simulink model "QD2_DroneStack_MPC"  (R2023a)
settings: Solver=ode1  StartTime=0.0  StopTime=inf  FixedStep=1/1000  RelTol=1e-3  EnableMultiTasking=on
InitFcn:
  | % QD2_DroneStack_MPC: rutas de la librería qd2_* y del mapeo de motores
  | qd2_d = fileparts(get_param(bdroot, 'FileName'));
  | for qd2_k = 1:4
  |     if exist(fullfile(qd2_d, 'lib', 'qd2_params.m'), 'file'), break; end
  |     qd2_d = fileparts(qd2_d);
  | end
  | addpath(fullfile(qd2_d, 'lib'));
  | addpath(fullfile(qd2_d, 'equipo2_original'));
  | clear qd2_d qd2_k
  | Motor_Mapping_7_Inch
model workspace (MAT data in the model file):
  target_system = 1
undefined symbols (not defined in the file): _Commander, _QDrone2, _Stabilizer, datetime, HIL, KT, lf, log_, m, Motor_Matrix, n, qc_get_step_size, s, saved_data
libraries: quarc_library x94, simulink x27, simulink_extras x9
(part 3 of 5)

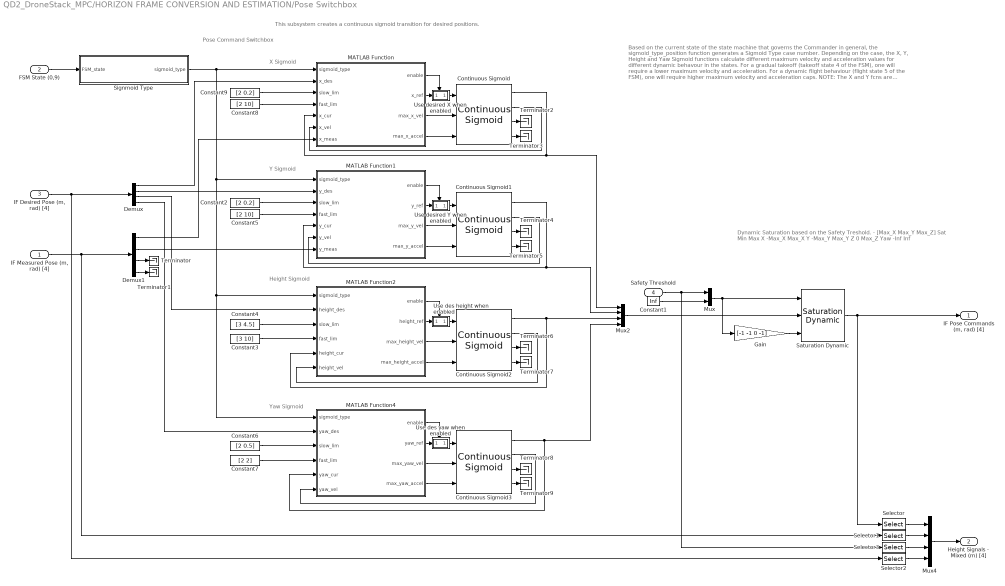
== system QD2_DroneStack_MPC/HORIZON FRAME CONVERSION AND ESTIMATION/Pose Switchbox ==
  note: Dynamic Saturation based on the Safety Treshold. - [Max_X Max_Y Max_Z]
      |
      | Sat Min Max
      | X -Max_X Max_X
      | Y -Max_Y Max_Y
      | Z 0 Max_Z
      | Yaw -Inf Inf
  note: Based on the current state of the state machine that governs the Commander in general,
      | the sigmoid_type_position function generates a Sigmoid Type case number. Depending on
      | the case, the X, Y, Height and Yaw Sigmoid functions calculate different maximum velocity
      | and acceleration values for different dynamic behavour in the states.
      |
      | For a gradual takeoff (takeoff state 4 of the FSM), one will require a lower maximum velocity
      | and acceleration. For a dynamic flight behaviour (flight state 5 of the FSM), one will require
      | higher maximum velocity and acceleration caps.
      |
      | NOTE: The X and Y fcns are logically identical due to the generally symmetric X and Y behaviour.
      | The Z and Yaw fcns are different.
  note: This subsystem creates a continuous sigmoid transition for desired positions.
  note: Height Sigmoid
  note: Pose Command Switchbox
  note: X Sigmoid
  note: Yaw Sigmoid
  note: Y Sigmoid
  "IF Measured Pose (m, rad) [4]" : Inport
  FSM State (0,9) : Inport  Port=2
  "IF Desired Pose (m, rad) [4]" : Inport  Port=3
  Safety Threshold : Inport  Port=4
  Constant1 : Constant  Value=Inf
  Constant2 : Constant  Value=[2 0.2]
  Constant3 : Constant  Value=[3 10]
  Constant4 : Constant  Value=[3 4.5]
  Constant5 : Constant  Value=[2 10]
  Constant6 : Constant  Value=[2 0.5]
  Constant7 : Constant  Value=[2 2]
  Constant8 : Constant  Value=[2 10]
  Constant9 : Constant  Value=[2 0.2]
  Continuous Sigmoid{,1..3} (4 alike) : quarc_library/Sources/Sigmoids/Continuous Sigmoid  params_source=External (input ports)  max_velocity=2  max_acceleration=10  initial_position=0  initial_velocity=0  hold_off=0.5  input_sample_time=-1  output_sample_time=qc_get_step_size
      settings: SourceProductName=QUARC Targets
  Demux : Demux
  Demux1 : Demux
  Gain : Gain  Gain=[-1 -1 0 -1]
  MATLAB Function : MATLAB Function  TreatAsAtomicUnit=on
  MATLAB Function1 : MATLAB Function  TreatAsAtomicUnit=on
  MATLAB Function2 : MATLAB Function  TreatAsAtomicUnit=on
  MATLAB Function4 : MATLAB Function  TreatAsAtomicUnit=on
  Mux : Mux  Inputs=2
  Mux2 : Mux
  Mux4 : Mux
  Saturation Dynamic : simulink/Discontinuities/Saturation Dynamic  OutMin=[]  OutMax=[]  OutDataTypeStr=Inherit: Same as second input  OutDataType=fixdt(1, 16)  OutScaling=2^-10  DoSatur=off
  Selector : Selector  InputPortWidth=4  IndexOptions=Index vector (dialog)  Indices=[3]  OutputSizes=1
  Selector1 : Selector  InputPortWidth=4  IndexOptions=Index vector (dialog)  Indices=[3]  OutputSizes=1
  Selector2 : Selector  InputPortWidth=4  IndexOptions=Index vector (dialog)  Indices=[3]  OutputSizes=1
  Selector3 : Selector  InputPortWidth=3  IndexOptions=Index vector (dialog)  Indices=[3]  OutputSizes=1
  Signmoid Type : MATLAB Function  TreatAsAtomicUnit=on
  Terminator{,1..9} (10 alike) : Terminator
  Use des height when enabled : Subsystem  TreatAsAtomicUnit=on
  Use des yaw when enabled : Subsystem  TreatAsAtomicUnit=on
  Use desired X when enabled : Subsystem  TreatAsAtomicUnit=on
  Use desired Y when enabled : Subsystem  TreatAsAtomicUnit=on
  "IF Pose Commands (m, rad) [4]" : Outport  VectorParamsAs1DForOutWhenUnconnected=off
  Height Signals - Mixed (m) [4] : Outport  Port=2  VectorParamsAs1DForOutWhenUnconnected=off
  wires:
  Constant4/1 -> MATLAB Function2/3(slow_lim)
  Constant3/1 -> MATLAB Function2/4(fast_lim)
  Selector/1 -> Mux4/1
  Selector1/1 -> Mux4/2
  Selector2/1 -> Mux4/4
  Selector3/1 -> Mux4/3
  Safety Threshold/1 -> Mux/1, Selector3/1
  Mux/1 -> Saturation Dynamic/1, Gain/1
  Constant1/1 -> Mux/2
  Saturation Dynamic/1 -> "IF Pose Commands (m, rad) [4]"/1, Selector/1
  Mux2/1 -> Saturation Dynamic/2
  Mux4/1 -> Height Signals - Mixed (m) [4]/1
  Gain/1 -> Saturation Dynamic/3
  Demux/2 -> MATLAB Function1/2(y_des)
  Use desired Y when enabled/1(Out1) -> Continuous Sigmoid1/1
  Use desired X when enabled/1(Out1) -> Continuous Sigmoid/1
  MATLAB Function2/3(max_height_vel) -> Continuous Sigmoid2/2
  Continuous Sigmoid3/3 -> Terminator8/1
  Demux1/4 -> Terminator1/1
  MATLAB Function4/1(enable) -> Use des yaw when enabled/Enable
  Use des yaw when enabled/1(Out1) -> Continuous Sigmoid3/1
  Continuous Sigmoid1/2 -> MATLAB Function1/6(y_vel)
  Constant2/1 -> MATLAB Function1/3(slow_lim)
  Constant6/1 -> MATLAB Function4/3(slow_lim)
  Demux1/1 -> MATLAB Function/7(x_meas)
  MATLAB Function1/2(y_ref) -> Use desired Y when enabled/1(h_d (m) [1])
  Demux/3 -> MATLAB Function2/2(height_des)
  Constant7/1 -> MATLAB Function4/4(fast_lim)
  Continuous Sigmoid1/4 -> Terminator5/1
  MATLAB Function1/1(enable) -> Use desired Y when enabled/Enable
  Continuous Sigmoid2/4 -> Terminator7/1
  Demux1/3 -> Terminator/1
  Signmoid Type/1(sigmoid_type) -> MATLAB Function/1(sigmoid_type), MATLAB Function1/1(sigmoid_type), MATLAB Function2/1(sigmoid_type), MATLAB Function4/1(sigmoid_type)
  MATLAB Function/3(max_x_vel) -> Continuous Sigmoid/2
  MATLAB Function2/1(enable) -> Use des height when enabled/Enable
  Constant9/1 -> MATLAB Function/3(slow_lim)
  Continuous Sigmoid2/2 -> MATLAB Function2/6(height_vel)
  Continuous Sigmoid1/1 -> MATLAB Function1/5(y_cur), Mux2/2
  MATLAB Function4/4(max_yaw_accel) -> Continuous Sigmoid3/3
  Demux/1 -> MATLAB Function/2(x_des)
  MATLAB Function1/3(max_y_vel) -> Continuous Sigmoid1/2
  Continuous Sigmoid3/2 -> MATLAB Function4/6(yaw_vel)
  MATLAB Function2/2(height_ref) -> Use des height when enabled/1(h_d (m) [1])
  MATLAB Function/4(max_x_accel) -> Continuous Sigmoid/3
  Use des height when enabled/1(Out1) -> Continuous Sigmoid2/1
  Continuous Sigmoid2/3 -> Terminator6/1
  Demux/4 -> MATLAB Function4/2(yaw_des)
  MATLAB Function1/4(max_y_accel) -> Continuous Sigmoid1/3
  MATLAB Function/1(enable) -> Use desired X when enabled/Enable
  Continuous Sigmoid3/4 -> Terminator9/1
  MATLAB Function4/2(yaw_ref) -> Use des yaw when enabled/1(h_d (m) [1])
  FSM State (0,9)/1 -> Signmoid Type/1(FSM_state)
  MATLAB Function2/4(max_height_accel) -> Continuous Sigmoid2/3
  Continuous Sigmoid/4 -> Terminator3/1
  Continuous Sigmoid/3 -> Terminator2/1
  Continuous Sigmoid/1 -> MATLAB Function/5(x_cur), Mux2/1
  Continuous Sigmoid/2 -> MATLAB Function/6(x_vel)
  MATLAB Function/2(x_ref) -> Use desired X when enabled/1(h_d (m) [1])
  Continuous Sigmoid3/1 -> MATLAB Function4/5(yaw_cur), Mux2/4
  MATLAB Function4/3(max_yaw_vel) -> Continuous Sigmoid3/2
  Continuous Sigmoid2/1 -> MATLAB Function2/5(height_cur), Mux2/3
  Demux1/2 -> MATLAB Function1/7(y_meas)
  Continuous Sigmoid1/3 -> Terminator4/1
  "IF Measured Pose (m, rad) [4]"/1 -> Demux1/1, Selector1/1
  "IF Desired Pose (m, rad) [4]"/1 -> Demux/1, Selector2/1
  Constant5/1 -> MATLAB Function1/4(fast_lim)
  Constant8/1 -> MATLAB Function/4(fast_lim)

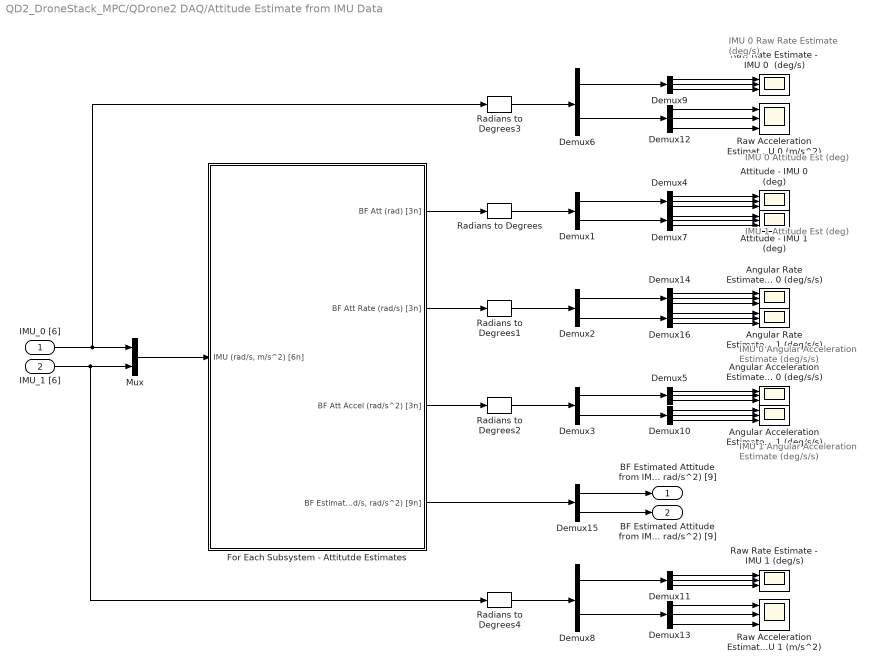
== system QD2_DroneStack_MPC/QDrone2 DAQ/Attitude Estimate from IMU Data ==
  note: IMU 0
      | Attitude Est (deg)
  note: IMU 1
      | Attitude Est (deg)
  note: IMU 0
      | Angular Acceleration
      | Estimate (deg/s/s)
  note: IMU 1
      | Angular Acceleration
      | Estimate (deg/s/s)
  note: IMU 0
      | Raw Rate Estimate (deg/s)
  IMU_0 [6] : Inport
  IMU_1 [6] : Inport  Port=2
  Angular Acceleration Estimate - IMU 0 (deg/s/s) : Scope  NumInputPorts=3
  Angular Acceleration Estimate IMU 1 (deg/s/s) : Scope  NumInputPorts=3
  Angular Rate Estimate - IMU 0 (deg/s/s) : Scope  NumInputPorts=3
  Angular Rate Estimate IMU 1 (deg/s/s) : Scope  NumInputPorts=3
  Attitude - IMU 0 (deg) : Scope  NumInputPorts=3
  Attitude - IMU 1 (deg) : Scope  NumInputPorts=3
  Demux{1..3,6,8} (5 alike) : Demux  Outputs=[3, 3]
  Demux{4..5,7,9..14,16} (10 alike) : Demux  Outputs=3
  Demux15 : Demux  Outputs=[9, 9]
  For Each Subsystem - Attitutde Estimates : Subsystem  TreatAsAtomicUnit=on
  Mux : Mux  Inputs=2
  Radians to Degrees{,1..4} (5 alike) : simulink_extras/Transformations/Radians to Degrees
  Raw Acceleration Estimate - IMU 0 (m/s^2) : Scope  NumInputPorts=3
  Raw Acceleration Estimate - IMU 1 (m/s^2) : Scope  NumInputPorts=3
  Raw Rate Estimate - IMU 0  (deg/s) : Scope  NumInputPorts=3
  Raw Rate Estimate - IMU 1 (deg/s) : Scope  NumInputPorts=3
  "BF Estimated Attitude from IMU 0 (rad, rad/s, rad/s^2) [9]" : Outport
  "BF Estimated Attitude from IMU 1 (rad, rad/s, rad/s^2) [9]" : Outport  Port=2
  wires:
  IMU_0 [6]/1 -> Radians to Degrees3/1, Mux/1
  IMU_1 [6]/1 -> Radians to Degrees4/1, Mux/2
  Mux/1 -> For Each Subsystem - Attitutde Estimates/1("IMU (rad/s, m/s^2) [6n]")
  For Each Subsystem - Attitutde Estimates/4("BF Estimated Att (rad, rad/s, rad/s^2) [9n] ") -> Demux15/1
  Demux15/1 -> "BF Estimated Attitude from IMU 0 (rad, rad/s, rad/s^2) [9]"/1
  Demux15/2 -> "BF Estimated Attitude from IMU 1 (rad, rad/s, rad/s^2) [9]"/1
  For Each Subsystem - Attitutde Estimates/1(BF Att (rad) [3n]) -> Radians to Degrees/1
  Radians to Degrees/1 -> Demux1/1
  For Each Subsystem - Attitutde Estimates/2(BF Att Rate (rad/s) [3n]) -> Radians to Degrees1/1
  For Each Subsystem - Attitutde Estimates/3(BF Att Accel (rad/s^2) [3n]) -> Radians to Degrees2/1
  Radians to Degrees1/1 -> Demux2/1
  Radians to Degrees2/1 -> Demux3/1
  Demux4/3 -> Attitude - IMU 0 (deg)/3
  Demux4/1 -> Attitude - IMU 0 (deg)/1
  Demux4/2 -> Attitude - IMU 0 (deg)/2
  Demux1/1 -> Demux4/1
  Demux7/2 -> Attitude - IMU 1 (deg)/2
  Demux7/1 -> Attitude - IMU 1 (deg)/1
  Demux7/3 -> Attitude - IMU 1 (deg)/3
  Demux1/2 -> Demux7/1
  Demux5/2 -> Angular Acceleration Estimate - IMU 0 (deg/s/s)/2
  Demux5/3 -> Angular Acceleration Estimate - IMU 0 (deg/s/s)/3
  Demux5/1 -> Angular Acceleration Estimate - IMU 0 (deg/s/s)/1
  Demux3/1 -> Demux5/1
  Demux10/1 -> Angular Acceleration Estimate IMU 1 (deg/s/s)/1
  Demux10/2 -> Angular Acceleration Estimate IMU 1 (deg/s/s)/2
  Demux10/3 -> Angular Acceleration Estimate IMU 1 (deg/s/s)/3
  Demux3/2 -> Demux10/1
  Demux12/2 -> Raw Acceleration Estimate - IMU 0 (m/s^2)/2
  Demux12/3 -> Raw Acceleration Estimate - IMU 0 (m/s^2)/3
  Demux12/1 -> Raw Acceleration Estimate - IMU 0 (m/s^2)/1
  Demux8/2 -> Demux13/1
  Demux13/2 -> Raw Acceleration Estimate - IMU 1 (m/s^2)/2
  Demux13/3 -> Raw Acceleration Estimate - IMU 1 (m/s^2)/3
  Demux13/1 -> Raw Acceleration Estimate - IMU 1 (m/s^2)/1
  Demux9/2 -> Raw Rate Estimate - IMU 0  (deg/s)/2
  Demux9/1 -> Raw Rate Estimate - IMU 0  (deg/s)/1
  Demux9/3 -> Raw Rate Estimate - IMU 0  (deg/s)/3
  Demux6/2 -> Demux12/1
  Demux6/1 -> Demux9/1
  Radians to Degrees3/1 -> Demux6/1
  Radians to Degrees4/1 -> Demux8/1
  Demux11/1 -> Raw Rate Estimate - IMU 1 (deg/s)/1
  Demux11/2 -> Raw Rate Estimate - IMU 1 (deg/s)/2
  Demux11/3 -> Raw Rate Estimate - IMU 1 (deg/s)/3
  Demux8/1 -> Demux11/1
  Demux2/2 -> Demux16/1
  Demux16/3 -> Angular Rate Estimate IMU 1 (deg/s/s)/3
  Demux16/1 -> Angular Rate Estimate IMU 1 (deg/s/s)/1
  Demux16/2 -> Angular Rate Estimate IMU 1 (deg/s/s)/2
  Demux2/1 -> Demux14/1
  Demux14/2 -> Angular Rate Estimate - IMU 0 (deg/s/s)/2
  Demux14/1 -> Angular Rate Estimate - IMU 0 (deg/s/s)/1
  Demux14/3 -> Angular Rate Estimate - IMU 0 (deg/s/s)/3

== system QD2_DroneStack_MPC/QDrone2 DAQ/Check Battery level ==
  Battery level : Inport
  Compare To Constant : simulink/Logic and Bit Operations/Compare To Constant  relop=<=  const=14  OutDataTypeStr=boolean
  Compare To Constant1 : simulink/Logic and Bit Operations/Compare To Constant  relop=>  const=0.5  OutDataTypeStr=boolean
  Data Type Conversion : DataTypeConversion  SaturateOnIntegerOverflow=off  RndMeth=Floor
  Data Type Conversion1 : DataTypeConversion  SaturateOnIntegerOverflow=off  RndMeth=Floor
  Logical Operator : Logic  AllPortsSameDT=off  OutDataTypeStr=boolean
  Terminator : Terminator
  Threshold : quarc_library/Discontinuities/Threshold  operator=>=  param_src=Specify via dialog  threshold=0.5  duration=0.3
      settings: SourceProductName=QUARC Targets
  Triggered Subsystem : Subsystem  TreatAsAtomicUnit=on
  Low Battery : Outport  VectorParamsAs1DForOutWhenUnconnected=off
  wires:
  Threshold/2 -> Terminator/1
  Battery level/1 -> Compare To Constant1/1, Compare To Constant/1
  Threshold/1 -> Logical Operator/2
  Logical Operator/1 -> Triggered Subsystem/Trigger
  Compare To Constant1/1 -> Logical Operator/1
  Compare To Constant/1 -> Data Type Conversion/1
  Data Type Conversion/1 -> Threshold/1
  Data Type Conversion1/1 -> Low Battery/1
  Triggered Subsystem/1(Out1) -> Data Type Conversion1/1

== system QD2_DroneStack_MPC/QDrone2 DAQ/Choose Motor Telemetry ==
  Bias1 : Bias  Bias=0:3  SaturateOnIntegerOverflow=off
  Constant : Constant  Value=[0 0 0 0; 0 0 0 1; 0 0 0 0; 0 0 1 0; 0 0 0 0; 0 1 0 0; 0 0 0 0; 1 0 0 0]
  Counter Free-Running : simulink/Sources/Counter Free-Running  NumBits=3  tsamp=-1
  Gain : Gain  Gain=.7
  Selector : Selector  NumberOfDimensions=2  IndexMode=Zero-based  InputPortWidth=3  IndexOptions=Index vector (port),Select all  Indices=[1 3],1  OutputSizes=1,1
  Telemetry : Scope
  Motor telemetry : Outport
  wires:
  Gain/1 -> Bias1/1
  Bias1/1 -> Telemetry/1
  Constant/1 -> Selector/1
  Counter Free-Running/1 -> Selector/2
  Selector/1 -> Motor telemetry/1, Gain/1

== system QD2_DroneStack_MPC/QDrone2 DAQ/Choose Motor Telemetry1 ==
  Channel : Inport
  Constant1 : Constant  Value=[1 0 0 0]
  Constant2 : Constant  Value=[0 1 0 0]
  Constant3 : Constant  Value=[0 0 1 0]
  Constant4 : Constant  Value=[0 0 0 1]
  Multiport Switch : MultiPortSwitch  DataPortOrder=Zero-based contiguous  Inputs=4  zeroidx=on  SaturateOnIntegerOverflow=off  InputSameDT=off
  Motor selection : Outport
  wires:
  Multiport Switch/1 -> Motor selection/1
  Constant4/1 -> Multiport Switch/5
  Constant3/1 -> Multiport Switch/4
  Constant1/1 -> Multiport Switch/2
  Constant2/1 -> Multiport Switch/3
  Channel/1 -> Multiport Switch/1

== system QD2_DroneStack_MPC/QDrone2 DAQ/Sensor Failure Monitoring - IMU0 ==
  note: Check for no data condition (flat-line zero) from any of the onboard sensors
  Sensor Data (rad/s,m/s^2)  [6] : Inport
  Data Type Conversion1 : DataTypeConversion  SaturateOnIntegerOverflow=off  RndMeth=Floor
  Data Type Conversion2 : DataTypeConversion  SaturateOnIntegerOverflow=off  RndMeth=Floor
  Data Type Conversion4 : DataTypeConversion  SaturateOnIntegerOverflow=off  RndMeth=Floor
  Demux : Demux  Outputs=[3 3]
  Logical Operator : Logic  Operator=OR  Inputs=1  AllPortsSameDT=off  OutDataTypeStr=boolean
  Mux : Mux  Inputs=2
  Sensor Failure (Accelerometer) : Subsystem
  Sensor Failure (Gyroscope) : Subsystem
  IMU Failure : Outport  VectorParamsAs1DForOutWhenUnconnected=off
  wires:
  Data Type Conversion4/1 -> IMU Failure/1
  Logical Operator/1 -> Data Type Conversion4/1
  Demux/1 -> Sensor Failure (Gyroscope)/1(Sensor Input)
  Data Type Conversion1/1 -> Mux/2
  Data Type Conversion2/1 -> Mux/1
  Mux/1 -> Logical Operator/1
  Sensor Failure (Accelerometer)/1(Sensor Fault) -> Data Type Conversion1/1
  Sensor Failure (Gyroscope)/1(Sensor Fault) -> Data Type Conversion2/1
  Demux/2 -> Sensor Failure (Accelerometer)/1(Sensor Input)
  Sensor Data (rad/s,m/s^2)  [6]/1 -> Demux/1

== system QD2_DroneStack_MPC/QDrone2 DAQ/Sensor Failure Monitoring - IMU1 ==
  note: Check for no data condition (flat-line zero) from any of the onboard sensors
  Sensor Data (rad/s,m/s^2)  [6] : Inport
  Data Type Conversion1 : DataTypeConversion  SaturateOnIntegerOverflow=off  RndMeth=Floor
  Data Type Conversion2 : DataTypeConversion  SaturateOnIntegerOverflow=off  RndMeth=Floor
  Data Type Conversion4 : DataTypeConversion  SaturateOnIntegerOverflow=off  RndMeth=Floor
  Demux : Demux  Outputs=[3 3]
  Logical Operator : Logic  Operator=OR  Inputs=1  AllPortsSameDT=off  OutDataTypeStr=boolean
  Mux : Mux  Inputs=2
  Sensor Failure (Accelerometer) : Subsystem
  Sensor Failure (Gyroscope) : Subsystem
  IMU Failure : Outport  VectorParamsAs1DForOutWhenUnconnected=off
  wires:
  Sensor Data (rad/s,m/s^2)  [6]/1 -> Demux/1
  Demux/2 -> Sensor Failure (Accelerometer)/1(Sensor Input)
  Sensor Failure (Gyroscope)/1(Sensor Fault) -> Data Type Conversion2/1
  Sensor Failure (Accelerometer)/1(Sensor Fault) -> Data Type Conversion1/1
  Mux/1 -> Logical Operator/1
  Data Type Conversion2/1 -> Mux/1
  Data Type Conversion1/1 -> Mux/2
  Demux/1 -> Sensor Failure (Gyroscope)/1(Sensor Input)
  Logical Operator/1 -> Data Type Conversion4/1
  Data Type Conversion4/1 -> IMU Failure/1

== system QD2_DroneStack_MPC/QDrone2 DAQ/Subsystem ==
  note: PCB LED 2
  note: PCB LED 1
  E_Stop (0,1) : Inport
  "Arm(0,1) " : Inport  Port=2
  Battery_State (bool) : Inport  Port=3
  Blue : Constant  Value=[0 0 1]
  Green : Constant  Value=[0 1 0]
  MATLAB Function LED Color Assignment : MATLAB Function  TreatAsAtomicUnit=on
  Multiport Switch : MultiPortSwitch  SaturateOnIntegerOverflow=off  InputSameDT=off
  Mux : Mux  Inputs=2
  Red : Constant  Value=[1 0 0]
  LEDs(%) [6] : Outport
  wires:
  Mux/1 -> LEDs(%) [6]/1
  Multiport Switch/1 -> Mux/1, Mux/2
  Blue/1 -> Multiport Switch/4
  Green/1 -> Multiport Switch/3
  Red/1 -> Multiport Switch/2
  Battery_State (bool)/1 -> MATLAB Function LED Color Assignment/3(low_battery)
  E_Stop (0,1)/1 -> MATLAB Function LED Color Assignment/1(E_Stop)
  "Arm(0,1) "/1 -> MATLAB Function LED Color Assignment/2(Arm)
  MATLAB Function LED Color Assignment/1(value) -> Multiport Switch/1

== system QD2_DroneStack_MPC/QDrone2 DAQ/Subsystem1 ==
  ESC % : Inport
  Motor command : Inport  Port=2
  Demux1 : Demux
  Demux3 : Demux
  Maintain previous value4 : Subsystem
  Mux{,1..3} (4 alike) : Mux  Inputs=2
  Selector : Selector  InputPortWidth=4  IndexOptions=Index vector (dialog)  Indices=[4 3 2 1]  OutputSizes=1
  Selector1 : Selector  InputPortWidth=4  IndexOptions=Index vector (dialog)  Indices=[4 3 2 1]  OutputSizes=1
  Out1 : Outport
  Out2 : Outport  Port=2
  Out3 : Outport  Port=3
  Out4 : Outport  Port=4
  wires:
  Motor command/1 -> Selector/1
  Demux1/2 -> Mux1/1
  Selector/1 -> Demux1/1
  Demux1/1 -> Mux/1
  Demux1/4 -> Mux3/1
  Demux1/3 -> Mux2/1
  Mux3/1 -> Out4/1
  Mux2/1 -> Out3/1
  Mux/1 -> Out1/1
  Mux1/1 -> Out2/1
  ESC %/1 -> Selector1/1
  Demux3/1 -> Mux/2
  Demux3/2 -> Mux1/2
  Demux3/3 -> Mux2/2
  Demux3/4 -> Mux3/2
  Selector1/1 -> Maintain previous value4/1(Value in)
  Maintain previous value4/1(Non 0 values) -> Demux3/1

== system QD2_DroneStack_MPC/STABILIZER - QDRONE 2/FLIGHT SAFETY ==
  note: If the watchdog times out, stop the model. This will shut off the motors as well.
  note: If communication with the model supplying reference commands has been lost for some time while the drone is armed, stop the model. This will shut off the motors as well.
  note: If the model supplying reference commands triggers a STOP MODEL command, stop this model. This will shut off the motors as well.
  note: Log Computation Time. This must be less than 0.001 s
  note: Log Sample Time. This must be approximately 0.001 s
  note: Flight Safety Information
      |
      | When a warning/stop message pops up, this is the subsystem
      | that generates them.
      |
      | Monitor Sample/Computation Time
      | Stop this model
      | when Stop Model is generated
      | communication loss is detected
      | Also log the watchdog monitor output
  Arm : Inport
  Stop Model : Inport  Port=2
  Communication Loss : Inport  Port=3
  Communication : quarc_library/Discontinuities/Threshold  operator=>=  param_src=Specify via dialog  threshold=0.5  duration=1
      settings: SourceProductName=QUARC Targets
  Computation Time : quarc_library/Sources/Time/Computation Time  sample_time=qc_get_step_size  use_model=on  use_cpu_time=off
  Computation Time (s) : Scope
  Data Type Conversion1 : DataTypeConversion  SaturateOnIntegerOverflow=off  RndMeth=Floor
  Data Type Conversion3 : DataTypeConversion  OutDataTypeStr=double  SaturateOnIntegerOverflow=off  RndMeth=Floor
  Data Type Conversion4 : DataTypeConversion  SaturateOnIntegerOverflow=off  RndMeth=Floor
  Data Type Conversion5 : DataTypeConversion  SaturateOnIntegerOverflow=off  RndMeth=Floor
  HIL Watchdog : quarc_library/Data Acquisition/Generic/Watchdog/HIL Watchdog  object_name=HIL-1  timeout=0.1  sample_time=qc_get_step_size  active=off
      settings: AttributesFormatString=(%<object_name>)  SourceProductName=QUARC Targets
  Logical Operator1 : Logic  AllPortsSameDT=off  OutDataTypeStr=boolean
  Mux : Mux
  Mux1 : Mux  Inputs=2
  Sample Time : quarc_library/Sources/Time/Sample Time  Priority=-99  sample_time=qc_get_step_size
  Sample Time (s) : Scope
  Stop model : quarc_library/Discontinuities/Threshold  operator=>=  param_src=Specify via dialog  threshold=0.5  duration=0.1
      settings: SourceProductName=QUARC Targets
  Stop with Message : quarc_library/Sinks/Error Handling/Stop with Message  message_type=Fixed error message  message_icon=Information  message=QDrone Stabilizer: Commander Terminated
  Stop with Message1 : quarc_library/Sinks/Error Handling/Stop with Message  message_type=Fixed error message  message_icon=Warning  message=QDrone Stabilizer: Communication with Commander lost
  Stop with Message3 : quarc_library/Sinks/Error Handling/Stop with Message  message_type=Fixed error message  message_icon=Information  message=QDrone Stabilizer: HIL Watchdog timer expired
  Terminator : Terminator
  Terminator1 : Terminator
  Safety Log : Outport  VectorParamsAs1DForOutWhenUnconnected=off
  wires:
  Data Type Conversion5/1 -> Mux/4
  Mux1/1 -> Mux/1
  Communication Loss/1 -> Logical Operator1/1
  Data Type Conversion3/1 -> Communication/1
  Communication/1 -> Stop with Message1/1, Data Type Conversion1/1
  Arm/1 -> Logical Operator1/2
  Data Type Conversion1/1 -> Mux/3
  Logical Operator1/1 -> Data Type Conversion3/1
  Communication/2 -> Terminator1/1
  Stop Model/1 -> Stop model/1
  Stop model/1 -> Stop with Message/1, Data Type Conversion4/1
  Stop model/2 -> Terminator/1
  HIL Watchdog/1 -> Data Type Conversion5/1, Stop with Message3/1
  Data Type Conversion4/1 -> Mux/2
  Sample Time/1 -> Mux1/1, Sample Time (s)/1
  Computation Time/1 -> Mux1/2, Computation Time (s)/1
  Mux/1 -> Safety Log/1

== system QD2_DroneStack_MPC/COMMANDER (ANGLE MODE)/STATE MACHINE SIGNALS/Generate Extra Messages for Console ==
  time (s) : Inport
  Signal Triggers : Inport  Port=2
  Boolean Edge-Based Triggered Print : Subsystem  TreatAsAtomicUnit=on
  Matrix Concatenate : Concatenate  NumInputs=3  Mode=Multidimensional array  ConcatenateDimension=2
  String Constant12 : quarc_library/Strings/String Constant  string_value=DRONE DISARMED  evaluate_string=off  string_type=text  max_length=80  sample_time=inf  variable_size=off
      settings: AttributesFormatString="\"DRONE DISARMED\""  SourceProductName=QUARC Targets
  String Constant13 : quarc_library/Strings/String Constant  string_value=DRONE LANDING  evaluate_string=off  string_type=text  max_length=80  sample_time=inf  variable_size=off
      settings: AttributesFormatString="\"DRONE LANDING\""  SourceProductName=QUARC Targets
  String Constant16 : quarc_library/Strings/String Constant  string_value=INITIALIZATION FINISHED  evaluate_string=off  string_type=text  max_length=80  sample_time=inf  variable_size=off
      settings: AttributesFormatString="\"INITIALIZATION FINISHED\""  SourceProductName=QUARC Targets
  Terminator : Terminator
  wires:
  Boolean Edge-Based Triggered Print/1(Out1) -> Terminator/1
  String Constant13/1 -> Matrix Concatenate/3
  String Constant12/1 -> Matrix Concatenate/2
  String Constant16/1 -> Matrix Concatenate/1
  Signal Triggers/1 -> Boolean Edge-Based Triggered Print/1(Signal Enable)
  time (s)/1 -> Boolean Edge-Based Triggered Print/3(time (s))
  Matrix Concatenate/1 -> Boolean Edge-Based Triggered Print/2(Message)

== system QD2_DroneStack_MPC/COMMANDER (ANGLE MODE)/STATE MACHINE SIGNALS/Generate State Messages for Console ==
  time (s) : Inport
  DroneState [1-9] : Inport  Port=2
  Detect Change : simulink/Logic and Bit Operations/Detect Change  vinit=0  OutDataTypeStr=boolean
  Multiport Switch : MultiPortSwitch  Inputs=9  SaturateOnIntegerOverflow=off  InputSameDT=off
  String Constant1 : quarc_library/Strings/String Constant  string_value=DRONE ARMED  evaluate_string=off  string_type=text  max_length=80  sample_time=inf  variable_size=off
      settings: AttributesFormatString="\"DRONE ARMED\""  SourceProductName=QUARC Targets
  String Constant2 : quarc_library/Strings/String Constant  string_value=DRONE TAKEOFF THROTTLE  evaluate_string=off  string_type=text  max_length=80  sample_time=inf  variable_size=off
      settings: AttributesFormatString="\"DRONE TAKEOFF THROTTLE\""  SourceProductName=QUARC Targets
  String Constant3 : quarc_library/Strings/String Constant  string_value=DRONE TAKEOFF HEIGHT STATE  evaluate_string=off  string_type=text  max_length=80  sample_time=inf  variable_size=off
      settings: AttributesFormatString="\"DRONE TAKEOFF HEIGHT STATE\""  SourceProductName=QUARC Targets
  String Constant4 : quarc_library/Strings/String Constant  string_value=ERROR - DRONE EMERGENCY STOP  evaluate_string=off  string_type=text  max_length=80  sample_time=inf  variable_size=off
      settings: AttributesFormatString="\"ERROR - DRONE EMERGENCY STOP\""  SourceProductName=QUARC Targets
  String Constant5 : quarc_library/Strings/String Constant  string_value=DRONE IDLE - WAITING TO BE ARMED  evaluate_string=off  string_type=text  max_length=80  sample_time=inf  variable_size=off
      settings: AttributesFormatString="\"DRONE IDLE - WAITING TO BE ARMED\""  SourceProductName=QUARC Targets
  String Constant6 : quarc_library/Strings/String Constant  string_value=DRONE IS IN FLIGHT STATE  evaluate_string=off  string_type=text  max_length=80  sample_time=inf  variable_size=off
      settings: AttributesFormatString="\"DRONE IS IN FLIGHT STATE\""  SourceProductName=QUARC Targets
  String Constant7 : quarc_library/Strings/String Constant  string_value=EMERGENCY STOP WAS PRESSED ON JOYSTICK  evaluate_string=off  string_type=text  max_length=80  sample_time=inf  variable_size=off
      settings: AttributesFormatString="\"EMERGENCY STOP WAS PRESSED ON JOYSTICK\""  SourceProductName=QUARC Targets
  String Constant8 : quarc_library/Strings/String Constant  string_value=FLIGHT FINISHED DRONE IS DISABLED  evaluate_string=off  string_type=text  max_length=80  sample_time=inf  variable_size=off
      settings: AttributesFormatString="\"FLIGHT FINISHED DRONE IS DISABLED\""  SourceProductName=QUARC Targets
  String Constant9 : quarc_library/Strings/String Constant  string_value=DRONE IS AUTO LANDING  evaluate_string=off  string_type=text  max_length=80  sample_time=inf  variable_size=off
      settings: AttributesFormatString="\"DRONE IS AUTO LANDING\""  SourceProductName=QUARC Targets
  Triggered Subsystem : Subsystem  TreatAsAtomicUnit=on
  wires:
  Detect Change/1 -> Triggered Subsystem/Trigger
  String Constant5/1 -> Multiport Switch/2
  String Constant8/1 -> Multiport Switch/10
  String Constant7/1 -> Multiport Switch/9
  String Constant4/1 -> Multiport Switch/8
  String Constant9/1 -> Multiport Switch/7
  String Constant6/1 -> Multiport Switch/6
  String Constant3/1 -> Multiport Switch/5
  String Constant2/1 -> Multiport Switch/4
  String Constant1/1 -> Multiport Switch/3
  time (s)/1 -> Triggered Subsystem/2(Time (s))
  Multiport Switch/1 -> Triggered Subsystem/3(Message)
  DroneState [1-9]/1 -> Detect Change/1, Triggered Subsystem/1(Value), Multiport Switch/1

== system QD2_DroneStack_MPC/COMMANDER (ANGLE MODE)/STATE MACHINE SIGNALS/Generate Warning Messages for Console ==
  time (s) : Inport
  errors [8] : Inport  Port=2
  Boolean Value-Based Triggered Print : Subsystem  TreatAsAtomicUnit=on
  Matrix Concatenate : Concatenate  NumInputs=9  Mode=Multidimensional array  ConcatenateDimension=2
  String Constant : quarc_library/Strings/String Constant  string_value=Commander: Low Battery  evaluate_string=off  string_type=text  max_length=80  sample_time=inf  variable_size=off
      settings: AttributesFormatString="\"Commander: Low Battery\""  SourceProductName=QUARC Targets
  String Constant1 : quarc_library/Strings/String Constant  string_value=Commander: Sensor Failure  evaluate_string=off  string_type=text  max_length=80  sample_time=inf  variable_size=off
      settings: AttributesFormatString="\"Commander: Sensor Failure\""  SourceProductName=QUARC Targets
  String Constant2 : quarc_library/Strings/String Constant  string_value=Commander: Host Stream Issue / Problem with communication  evaluate_string=off  string_type=text  max_length=80  sample_time=inf  variable_size=off
      settings: AttributesFormatString="\"Commander: Host Stream Issue / Problem with communication\""  SourceProductName=QUARC Targets
  String Constant3 : quarc_library/Strings/String Constant  string_value=Commander: Joystick Issue  evaluate_string=off  string_type=text  max_length=80  sample_time=inf  variable_size=off
      settings: AttributesFormatString="\"Commander: Joystick Issue\""  SourceProductName=QUARC Targets
  String Constant4 : quarc_library/Strings/String Constant  string_value=Commander: Optitrack isn't tracking  evaluate_string=off  string_type=text  max_length=80  sample_time=inf  variable_size=off
      settings: AttributesFormatString="\"Commander: Optitrack isn't tracking\""  SourceProductName=QUARC Targets
  String Constant5 : quarc_library/Strings/String Constant  string_value=Commander: Flying low  evaluate_string=off  string_type=text  max_length=80  sample_time=inf  variable_size=off
      settings: AttributesFormatString="\"Commander: Flying low\""  SourceProductName=QUARC Targets
  String Constant6 : quarc_library/Strings/String Constant  string_value=Commander: Flying high  evaluate_string=off  string_type=text  max_length=80  sample_time=inf  variable_size=off
      settings: AttributesFormatString="\"Commander: Flying high\""  SourceProductName=QUARC Targets
  String Constant7 : quarc_library/Strings/String Constant  string_value=Commander: Emergency Stop Triggered  evaluate_string=off  string_type=text  max_length=80  sample_time=inf  variable_size=off
      settings: AttributesFormatString="\"Commander: Emergency Stop Triggered\""  SourceProductName=QUARC Targets
  String Constant8 : quarc_library/Strings/String Constant  string_value=Commander: Takeoff triggered before armed drone  evaluate_string=off  string_type=text  max_length=80  sample_time=inf  variable_size=off
      settings: AttributesFormatString="\"Commander: Takeoff triggered before armed drone\""  SourceProductName=QUARC Targets
  Terminator : Terminator
  wires:
  time (s)/1 -> Boolean Value-Based Triggered Print/3(time (s))
  errors [8]/1 -> Boolean Value-Based Triggered Print/1(Signal Enable)
  Matrix Concatenate/1 -> Boolean Value-Based Triggered Print/2(Message)
  String Constant/1 -> Matrix Concatenate/1
  String Constant1/1 -> Matrix Concatenate/2
  String Constant2/1 -> Matrix Concatenate/3
  String Constant3/1 -> Matrix Concatenate/4
  Boolean Value-Based Triggered Print/1(Out1) -> Terminator/1
  String Constant7/1 -> Matrix Concatenate/9
  String Constant6/1 -> Matrix Concatenate/8
  String Constant5/1 -> Matrix Concatenate/7
  String Constant4/1 -> Matrix Concatenate/6
  String Constant8/1 -> Matrix Concatenate/5

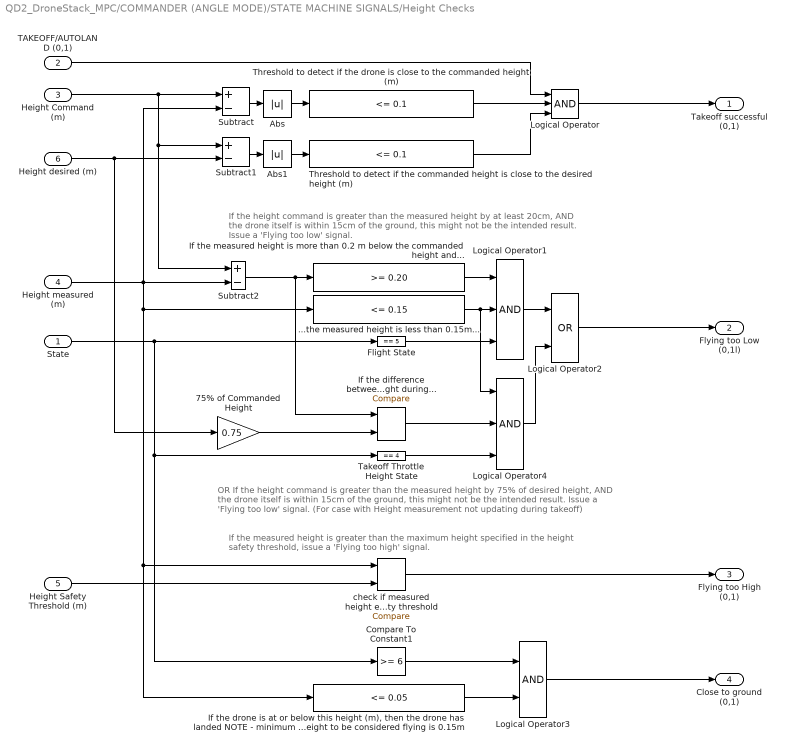
== system QD2_DroneStack_MPC/COMMANDER (ANGLE MODE)/STATE MACHINE SIGNALS/Height Checks ==
  note: If the height command is greater than the measured height by at least 20cm, AND the drone itself is
      | within 15cm of the ground, this might not be the intended result. Issue a 'Flying too low' signal.
  note: If the measured height is greater than the maximum height specified in the height safety threshold,
      | issue a 'Flying too high' signal.
  note: OR If the height command is greater than the measured height by 75% of desired height, AND
      | the drone itself is within 15cm of the ground, this might not be the intended result. Issue a 'Flying too low' signal.
      | (For case with Height measurement not updating during takeoff)
  State : Inport
  TAKEOFF/AUTOLAND (0,1) : Inport  Port=2
  Height Command (m) : Inport  Port=3
  Height measured (m) : Inport  Port=4
  Height Safety Threshold (m) : Inport  Port=5
  Height desired (m) : Inport  Port=6
  ...the measured height is less than 0.15m... : simulink/Logic and Bit Operations/Compare To Constant  relop=<=  const=0.15  OutDataTypeStr=boolean
  75% of Commanded Height : Gain  Gain=0.75
  Abs : Abs  SaturateOnIntegerOverflow=off
  Abs1 : Abs  SaturateOnIntegerOverflow=off
  Compare To Constant1 : simulink/Logic and Bit Operations/Compare To Constant  relop=>=  const=6  OutDataTypeStr=boolean
  Flight State : simulink/Logic and Bit Operations/Compare To Constant  relop===  const=5  OutDataTypeStr=boolean
  If the difference between the measured and commanded height is greater than 75% of the commanded height during... : quarc_library/Logic Operations/Compare  operator=>=  output_data_type=boolean
      settings: SourceProductName=QUARC Targets
  "If the drone is at or below this height (m), then the drone has landed NOTE - minimum height to be considered flying is 0.15m   " : simulink/Logic and Bit Operations/Compare To Constant  relop=<=  const=0.05  OutDataTypeStr=boolean
  If the measured height is more than 0.2 m below the commanded height and... : simulink/Logic and Bit Operations/Compare To Constant  relop=>=  const=0.20  OutDataTypeStr=boolean
  Logical Operator : Logic  Inputs=3  AllPortsSameDT=off  OutDataTypeStr=boolean
  Logical Operator1 : Logic  Inputs=3  AllPortsSameDT=off  OutDataTypeStr=boolean
  Logical Operator2 : Logic  Operator=OR  AllPortsSameDT=off  OutDataTypeStr=boolean
  Logical Operator3 : Logic  AllPortsSameDT=off  OutDataTypeStr=boolean
  Logical Operator4 : Logic  Inputs=3  AllPortsSameDT=off  OutDataTypeStr=boolean
  Subtract : Sum  Inputs=+-
  Subtract1 : Sum  Inputs=+-
  Subtract2 : Sum  Inputs=+-
  Takeoff Throttle Height State : simulink/Logic and Bit Operations/Compare To Constant  relop===  const=4  OutDataTypeStr=boolean
  Threshold to detect if the commanded height is close to the desired height (m) : simulink/Logic and Bit Operations/Compare To Constant  relop=<=  const=0.1  OutDataTypeStr=boolean
  Threshold to detect if the drone is close to the commanded height (m) : simulink/Logic and Bit Operations/Compare To Constant  relop=<=  const=0.1  OutDataTypeStr=boolean
  check if measured height exceeds maximum height safety threshold : quarc_library/Logic Operations/Compare  operator=>=  output_data_type=boolean
      settings: SourceProductName=QUARC Targets
  Takeoff successful (0,1) : Outport  VectorParamsAs1DForOutWhenUnconnected=off
  Flying too Low (0,1l) : Outport  Port=2  VectorParamsAs1DForOutWhenUnconnected=off
  Flying too High (0,1) : Outport  Port=3  VectorParamsAs1DForOutWhenUnconnected=off
  Close to ground (0,1) : Outport  Port=4  VectorParamsAs1DForOutWhenUnconnected=off
  wires:
  Logical Operator/1 -> Takeoff successful (0,1)/1
  Logical Operator2/1 -> Flying too Low (0,1l)/1
  Subtract1/1 -> Abs1/1
  Threshold to detect if the commanded height is close to the desired height (m)/1 -> Logical Operator/3
  Abs/1 -> Threshold to detect if the drone is close to the commanded height (m)/1
  Threshold to detect if the drone is close to the commanded height (m)/1 -> Logical Operator/2
  Abs1/1 -> Threshold to detect if the commanded height is close to the desired height (m)/1
  Height desired (m)/1 -> 75% of Commanded Height/1, Subtract1/2
  TAKEOFF/AUTOLAND (0,1)/1 -> Logical Operator/1
  Subtract/1 -> Abs/1
  If the measured height is more than 0.2 m below the commanded height and.../1 -> Logical Operator1/1
  Logical Operator1/1 -> Logical Operator2/1
  Height Command (m)/1 -> Subtract1/1, Subtract2/1, Subtract/1
  ...the measured height is less than 0.15m.../1 -> Logical Operator4/1, Logical Operator1/2
  check if measured height exceeds maximum height safety threshold/1 -> Flying too High (0,1)/1
  Height Safety Threshold (m)/1 -> check if measured height exceeds maximum height safety threshold/2
  State/1 -> Flight State/1, Takeoff Throttle Height State/1, Compare To Constant1/1
  Logical Operator3/1 -> Close to ground (0,1)/1
  "If the drone is at or below this height (m), then the drone has landed NOTE - minimum height to be considered flying is 0.15m   "/1 -> Logical Operator3/2
  Compare To Constant1/1 -> Logical Operator3/1
  Height measured (m)/1 -> Subtract/2, ...the measured height is less than 0.15m.../1, "If the drone is at or below this height (m), then the drone has landed NOTE - minimum height to be considered flying is 0.15m   "/1, check if measured height exceeds maximum height safety threshold/1, Subtract2/2
  Logical Operator4/1 -> Logical Operator2/2
  Flight State/1 -> Logical Operator1/3
  Subtract2/1 -> If the difference between the measured and commanded height is greater than 75% of the commanded height during.../1, If the measured height is more than 0.2 m below the commanded height and.../1
  Takeoff Throttle Height State/1 -> Logical Operator4/3
  75% of Commanded Height/1 -> If the difference between the measured and commanded height is greater than 75% of the commanded height during.../2
  If the difference between the measured and commanded height is greater than 75% of the commanded height during.../1 -> Logical Operator4/2

== system QD2_DroneStack_MPC/COMMANDER (ANGLE MODE)/STATE MACHINE SIGNALS/Latch E-Stop ==
  Input : Inport
  Trigger : TriggerPort  VariantControl=Variant
  Latched Output : Outport  InitialOutput=0  VectorParamsAs1DForOutWhenUnconnected=off
  wires:
  Input/1 -> Latched Output/1

== system QD2_DroneStack_MPC/COMMANDER (ANGLE MODE)/STATE MACHINE SIGNALS/Throttle Checks ==
  Throttle Command (N) : Inport
  Controller Throttle Command (N) : Inport  Port=2
  Throttle Trim (N) : Inport  Port=3
  Max Thrust (N) : Inport  Port=4
  Abs : Abs  SaturateOnIntegerOverflow=off
  Abs1 : Abs  SaturateOnIntegerOverflow=off
  Compare : quarc_library/Logic Operations/Compare  operator=<=  output_data_type=boolean
      settings: SourceProductName=QUARC Targets
  Compare1 : quarc_library/Logic Operations/Compare  operator=<=  output_data_type=boolean
      settings: SourceProductName=QUARC Targets
  Compare2 : quarc_library/Logic Operations/Compare  operator=<=  output_data_type=boolean
      settings: SourceProductName=QUARC Targets
  "MAX throttle percentage (%) For CMD " : Constant  Value=0.171
  "MAX throttle percentage (%) For Ctrl " : Constant  Value=0.068
  "MAX throttle percentage (%) For Trim  " : Constant  Value=0.034
  Product : Product
  Product1 : Product
  Product2 : Product
  Subtract : Sum  Inputs=+-
  Threshold below which throttle can be assumed to be close to zero (N) (17.1% of Max Thrust) : simulink/Logic and Bit Operations/Compare To Constant  Commented=on  relop=<=  const=3.5  OutDataTypeStr=boolean
  Threshold to determine if the controller throttle is close to zero (N) (6.8% of Max Thrust) : simulink/Logic and Bit Operations/Compare To Constant  Commented=on  relop=<=  const=1.40  OutDataTypeStr=boolean
  Threshold to determine if throttle is close to the trim value (N) (3.4% of Max Thrust) : simulink/Logic and Bit Operations/Compare To Constant  Commented=on  relop=<=  const=0.7  OutDataTypeStr=boolean
  CMD Throttle at Trim (0,1) : Outport  VectorParamsAs1DForOutWhenUnconnected=off
  CMD Throttle close to 0 (0,1) : Outport  Port=2  VectorParamsAs1DForOutWhenUnconnected=off
  Ctrl Throttle close to 0 (0,1) : Outport  Port=3  VectorParamsAs1DForOutWhenUnconnected=off
  wires:
  Throttle Command (N)/1 -> Compare1/1, Subtract/1
  Throttle Trim (N)/1 -> Subtract/2
  Subtract/1 -> Abs/1
  Compare/1 -> CMD Throttle at Trim (0,1)/1
  Compare1/1 -> CMD Throttle close to 0 (0,1)/1
  Abs1/1 -> Compare2/1
  Controller Throttle Command (N)/1 -> Abs1/1
  Compare2/1 -> Ctrl Throttle close to 0 (0,1)/1
  "MAX throttle percentage (%) For Trim  "/1 -> Product1/1
  "MAX throttle percentage (%) For CMD "/1 -> Product/1
  "MAX throttle percentage (%) For Ctrl "/1 -> Product2/1
  Max Thrust (N)/1 -> Product1/2, Product/2, Product2/2
  Product1/1 -> Compare/2
  Abs/1 -> Compare/1
  Product/1 -> Compare1/2
  Product2/1 -> Compare2/2

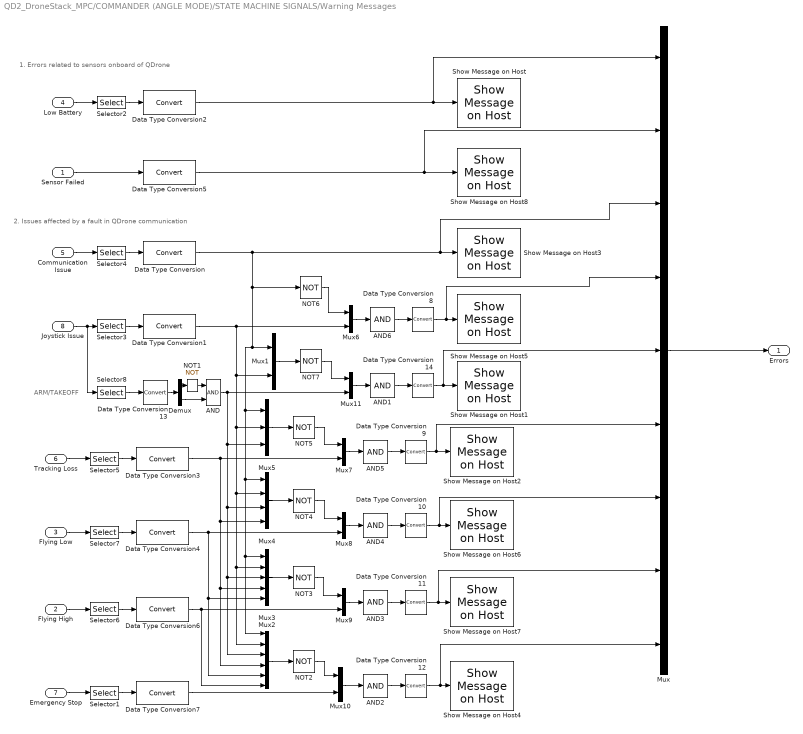
== system QD2_DroneStack_MPC/COMMANDER (ANGLE MODE)/STATE MACHINE SIGNALS/Warning Messages ==
  note: ARM/TAKEOFF
  note: 1. Errors related to sensors onboard of QDrone
  note: 2. Issues affected by a fault in QDrone communication
  Sensor Failed : Inport
  Flying High : Inport  Port=2
  Flying Low : Inport  Port=3
  Low Battery : Inport  Port=4
  Communication Issue : Inport  Port=5
  Tracking Loss : Inport  Port=6
  "Emergency Stop " : Inport  Port=7
  Joystick Issue : Inport  Port=8
  AND : Logic  AllPortsSameDT=off  OutDataTypeStr=boolean
  AND{1..6} (6 alike) : Logic  Inputs=1  AllPortsSameDT=off  OutDataTypeStr=boolean
  Data Type Conversion{,1..14} (15 alike) : DataTypeConversion  SaturateOnIntegerOverflow=off  RndMeth=Floor
  Demux : Demux  Outputs=2
  Mux : Mux  Inputs=9
  Mux1 : Mux  Inputs=[1 1]
  Mux{6..11} (6 alike) : Mux  Inputs=2
  Mux2 : Mux  Inputs=[1 1 1 1 1 1]
  Mux3 : Mux  Inputs=[ 1 1 1 1 1]
  Mux4 : Mux  Inputs=[1 1 1 1]
  Mux5 : Mux  Inputs=[1 1 1]
  NOT{1..7} (7 alike) : Logic  Operator=NOT  IconShape=distinctive  AllPortsSameDT=off  OutDataTypeStr=boolean
  Selector1 : Selector  InputPortWidth=4  IndexOptions=Index vector (dialog)  Indices=3  OutputSizes=1
  Selector2 : Selector  InputPortWidth=5  IndexOptions=Index vector (dialog)  Indices=5  OutputSizes=1
  Selector3 : Selector  InputPortWidth=4  IndexOptions=Index vector (dialog)  Indices=4  OutputSizes=1
  Selector4 : Selector  InputPortWidth=5  IndexOptions=Index vector (dialog)  Indices=4  OutputSizes=1
  Selector5 : Selector  InputPortWidth=5  IndexOptions=Index vector (dialog)  Indices=3  OutputSizes=1
  Selector6 : Selector  InputPortWidth=4  IndexOptions=Index vector (dialog)  Indices=3  OutputSizes=1
  Selector7 : Selector  InputPortWidth=4  IndexOptions=Index vector (dialog)  Indices=2  OutputSizes=1
  Selector8 : Selector  InputPortWidth=4  IndexOptions=Index vector (dialog)  Indices=[1:2]  OutputSizes=1
  Show Message on Host : quarc_library/Sinks/Error Handling/Show Message on Host  message_type=Fixed error message  message_icon=Warning  message=Commander: Low Battery
      settings: AttributesFormatString="\"%<message>\""  SourceProductName=QUARC Targets
  Show Message on Host1 : quarc_library/Sinks/Error Handling/Show Message on Host  message_type=Fixed error message  message_icon=Warning  message=Commander: Takeoff triggered before armed drone
      settings: AttributesFormatString="\"%<message>\""  SourceProductName=QUARC Targets
  Show Message on Host2 : quarc_library/Sinks/Error Handling/Show Message on Host  message_type=Fixed error message  message_icon=Warning  message=Commander: Optitrack isn't tracking
      settings: AttributesFormatString="\"%<message>\""  SourceProductName=QUARC Targets
  Show Message on Host3 : quarc_library/Sinks/Error Handling/Show Message on Host  message_type=Fixed error message  message_icon=Warning  message=Commander: Host Stream Issue
      settings: AttributesFormatString="\"%<message>\""  SourceProductName=QUARC Targets
  Show Message on Host4 : quarc_library/Sinks/Error Handling/Show Message on Host  message_type=Fixed error message  message_icon=Warning  message=Commander: Emergency Stop Triggered
      settings: AttributesFormatString="\"%<message>\""  SourceProductName=QUARC Targets
  Show Message on Host5 : quarc_library/Sinks/Error Handling/Show Message on Host  message_type=Fixed error message  message_icon=Warning  message=Commander: Joystick Issue
      settings: AttributesFormatString="\"%<message>\""  SourceProductName=QUARC Targets
  Show Message on Host6 : quarc_library/Sinks/Error Handling/Show Message on Host  message_type=Fixed error message  message_icon=Warning  message=Commander: Flying low
      settings: AttributesFormatString="\"%<message>\""  SourceProductName=QUARC Targets
  Show Message on Host7 : quarc_library/Sinks/Error Handling/Show Message on Host  message_type=Fixed error message  message_icon=Warning  message=Commander: Flying high
      settings: AttributesFormatString="\"%<message>\""  SourceProductName=QUARC Targets
  Show Message on Host8 : quarc_library/Sinks/Error Handling/Show Message on Host  message_type=Fixed error message  message_icon=Warning  message=Commander: Sensor Failure
      settings: AttributesFormatString="\"%<message>\""  SourceProductName=QUARC Targets
  Errors : Outport
  wires:
  NOT2/1 -> Mux10/1
  Mux2/1 -> NOT2/1
  NOT3/1 -> Mux9/1
  Mux3/1 -> NOT3/1
  NOT4/1 -> Mux8/1
  Mux4/1 -> NOT4/1
  NOT5/1 -> Mux7/1
  Mux5/1 -> NOT5/1
  NOT6/1 -> Mux6/1
  Sensor Failed/1 -> Data Type Conversion5/1
  Selector6/1 -> Data Type Conversion6/1
  Selector1/1 -> Data Type Conversion7/1
  Low Battery/1 -> Selector2/1
  Communication Issue/1 -> Selector4/1
  "Emergency Stop "/1 -> Selector1/1
  AND2/1 -> Data Type Conversion12/1
  AND3/1 -> Data Type Conversion11/1
  AND4/1 -> Data Type Conversion10/1
  AND5/1 -> Data Type Conversion9/1
  AND6/1 -> Data Type Conversion8/1
  Selector2/1 -> Data Type Conversion2/1
  Selector3/1 -> Data Type Conversion1/1
  Selector4/1 -> Data Type Conversion/1
  Selector5/1 -> Data Type Conversion3/1
  Selector7/1 -> Data Type Conversion4/1
  Data Type Conversion3/1 -> Mux7/2, Mux4/4, Mux3/4, Mux2/4
  Data Type Conversion4/1 -> Mux8/2, Mux2/5, Mux3/5
  Data Type Conversion6/1 -> Mux2/6, Mux9/2
  Data Type Conversion7/1 -> Mux10/2
  Mux6/1 -> AND6/1
  Mux10/1 -> AND2/1
  Data Type Conversion12/1 -> Mux/9, Show Message on Host4/1
  Mux9/1 -> AND3/1
  Mux7/1 -> AND5/1
  Mux8/1 -> AND4/1
  Data Type Conversion2/1 -> Mux/1, Show Message on Host/1
  Data Type Conversion5/1 -> Mux/2, Show Message on Host8/1
  Tracking Loss/1 -> Selector5/1
  Flying Low/1 -> Selector7/1
  Flying High/1 -> Selector6/1
  Joystick Issue/1 -> Selector8/1, Selector3/1
  Data Type Conversion9/1 -> Mux/6, Show Message on Host2/1
  Data Type Conversion8/1 -> Mux/4, Show Message on Host5/1
  Data Type Conversion10/1 -> Mux/7, Show Message on Host6/1
  Data Type Conversion11/1 -> Mux/8, Show Message on Host7/1
  Mux/1 -> Errors/1
  Selector8/1 -> Data Type Conversion13/1
  Data Type Conversion13/1 -> Demux/1
  Demux/1 -> NOT1/1
  Demux/2 -> AND/2
  NOT1/1 -> AND/1
  NOT7/1 -> Mux11/1
  Data Type Conversion14/1 -> Mux/5, Show Message on Host1/1
  AND1/1 -> Data Type Conversion14/1
  Data Type Conversion1/1 -> Mux6/2, Mux1/2, Mux5/2, Mux4/2, Mux3/2, Mux2/2
  Mux11/1 -> AND1/1
  Data Type Conversion/1 -> NOT6/1, Mux1/1, Mux5/1, Mux4/1, Mux3/1, Mux2/1, Mux/3, Show Message on Host3/1
  Mux1/1 -> NOT7/1
  AND/1 -> Mux2/3, Mux3/3, Mux4/3, Mux5/3, Mux11/2

== system QD2_DroneStack_MPC/COMMANDER (ANGLE MODE)/THROTTLE SWITCHBOX /Use desired height when enabled ==
  h_d (m) [1] : Inport
  Enable : EnablePort
  Out1 : Outport  OutputWhenDisabled=reset  InitialOutput=0  VectorParamsAs1DForOutWhenUnconnected=off
  wires:
  h_d (m) [1]/1 -> Out1/1

== system QD2_DroneStack_MPC/HORIZON FRAME CONVERSION AND ESTIMATION/Pose Switchbox/Use des height when enabled ==
  h_d (m) [1] : Inport
  Enable : EnablePort
  Out1 : Outport  OutputWhenDisabled=reset  InitialOutput=0  VectorParamsAs1DForOutWhenUnconnected=off
  wires:
  h_d (m) [1]/1 -> Out1/1

== system QD2_DroneStack_MPC/HORIZON FRAME CONVERSION AND ESTIMATION/Pose Switchbox/Use des yaw when enabled ==
  h_d (m) [1] : Inport
  Enable : EnablePort
  Out1 : Outport  OutputWhenDisabled=reset  InitialOutput=0  VectorParamsAs1DForOutWhenUnconnected=off
  wires:
  h_d (m) [1]/1 -> Out1/1

== system QD2_DroneStack_MPC/HORIZON FRAME CONVERSION AND ESTIMATION/Pose Switchbox/Use desired X when enabled ==
  h_d (m) [1] : Inport
  Enable : EnablePort
  Out1 : Outport  OutputWhenDisabled=reset  InitialOutput=0  VectorParamsAs1DForOutWhenUnconnected=off
  wires:
  h_d (m) [1]/1 -> Out1/1

== system QD2_DroneStack_MPC/HORIZON FRAME CONVERSION AND ESTIMATION/Pose Switchbox/Use desired Y when enabled ==
  h_d (m) [1] : Inport
  Enable : EnablePort
  Out1 : Outport  OutputWhenDisabled=reset  InitialOutput=0  VectorParamsAs1DForOutWhenUnconnected=off
  wires:
  h_d (m) [1]/1 -> Out1/1
